simulink model "ex_kloss_startup"  (R2026b)
settings: Solver=ode23t  StopTime=2  MaxStep=1e-4  RelTol=1e-5
libraries: asm_blocks_lib x11, nesl_utility x1
settings Model: Creator=fsbb  LastModifiedBy=fsbb
settings SimscapeCC: SimscapeLogType=all  SimscapeNominalValues="[{\"value\":\"1\",\"unit\":\"A\"},{\"value\":\"1\",\"unit\":\"bar\"},{\"value\":\"1\",\"unit\":\"cm^2\"},{\"value\":\"1\",\"unit\":\"cm^3/s\"},{\"value\":\"1\",\"unit\":\"kJ/kg\"},{\"value\":\"1\",\"unit\":\"kW\"},{\"value\":\"1\",\"unit\":\"l\"},{\"value\":\"1\",\"unit\":\"N\"},{\"value\":\"1\",\"unit\":\"N*m\"},{\"value\":\"1\",\"unit\":\"V\"},{\"value\":\"0.001\",\"unit\":\"Wb\"}]"  SimscapeUseEnergyAccounting=off

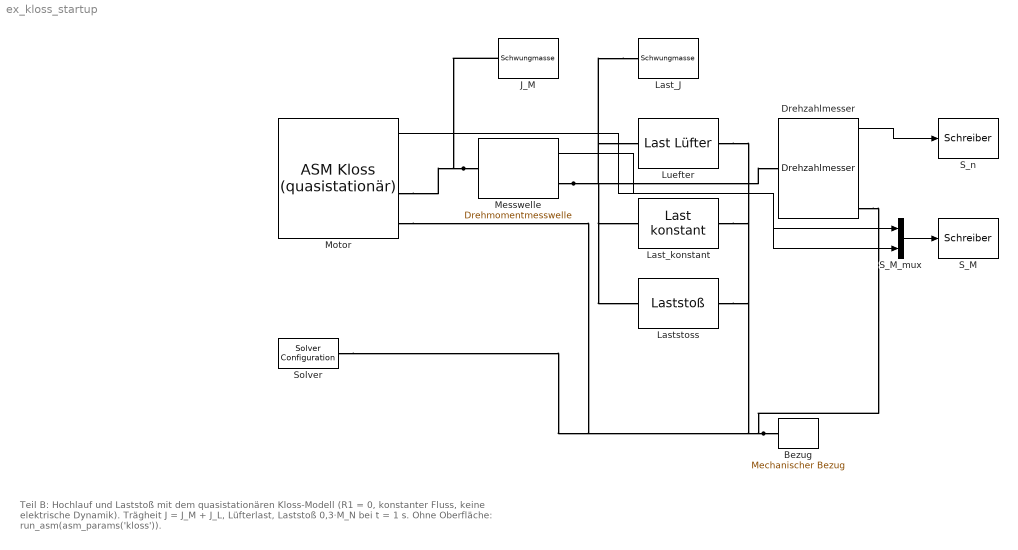
== system ex_kloss_startup ==
  note: Teil B: Hochlauf und Laststoß mit dem quasistationären Kloss-Modell (R1 = 0, konstanter Fluss, keine elektrische Dynamik). Trägheit J = J_M + J_L, Lüfterlast, Laststoß 0,3·M_N bei t = 1 s. Ohne Oberfläche: run_asm(asm_params('kloss')).
  Bezug : asm_blocks_lib/Mechanik/Mechanischer Bezug  Tag=asmlib:mech_reference
  Drehzahlmesser : asm_blocks_lib/Messgeräte/Drehzahlmesser  Tag=asmlib:speed_sensor  ns=1500
  J_M : asm_blocks_lib/Mechanik/Schwungmasse  Tag=asmlib:inertia  J=0.012  n0=0
  Last_J : asm_blocks_lib/Mechanik/Schwungmasse  Tag=asmlib:inertia  J=0.01  n0=0
  Last_konstant : asm_blocks_lib/Mechanik/Last konstant  Tag=asmlib:load_constant  M_L0=0
  Laststoss : asm_blocks_lib/Mechanik/Laststoß  Tag=asmlib:load_step  t_step=1  dM_L=7.95
  Luefter : asm_blocks_lib/Mechanik/Last Lüfter  Tag=asmlib:load_fan  M_B=26.5  n_B=1440
  Messwelle : asm_blocks_lib/Messgeräte/Drehmomentmesswelle  Tag=asmlib:torque_sensor
  Motor : asm_blocks_lib/Referenz/ASM Kloss (quasistationär)  Tag=asmlib:asm_kloss  MK=71.55  sK=0.2  ns=1500
  S_M : asm_blocks_lib/Messgeräte/Schreiber  Tag=asmlib:recorder  title_text=Motormoment (Kloss) und Wellenmoment
  S_M_mux : Mux  Inputs=2
  S_n : asm_blocks_lib/Messgeräte/Schreiber  Tag=asmlib:recorder  title_text=Drehzahl
  Solver : nesl_utility/Solver Configuration  PhysicalDomain=network_engine_domain  SubClassName=solver  LeftPortType=input  RightPortType=generic  Tones=[]  Harmonics=[]  SimulateNoise=off  Profile=off  UseLocalSampling=off  EnableSwitchedLinearOptims=on  FrequencyDomain=off  UseCCode=off  RelTol=0.001  AbsTol=0.001  MinStep=1e-09  ToWorkspace=off  RevertToSquareIcSolve=off  NumHomotopyIterations=100  PhasorMode=off  PhasorModeNumHarmonics=1  ConsistencySolver=NEWTON_XTOL_AFTER_FTOL  CanonicalOrdering=CANONICAL  OptimizeIntermediates=OPTIMIZED  MulticoreSolverChoice=BACKWARD_EULER  IndexReductionMethod=DerivativeReplacement  DoDC=off  ResidualTolerance=1e-09  ConsistencyTolSource=GLOBAL  ConsistencyAbsTol=0.001  ConsistencyRelTol=0.001  ConsistencyTolFactor=0.001  UseLocalSolver=off  LocalSolverChoice=NE_BACKWARD_EULER_ADVANCER  ResolveIndetEquations=on  FunctionEvalNumThread=1  LocalSolverSampleTime=0.001  DoFixedCost=off  MaxNonlinIter=3  MaxModeIter=2  ComputeImpulses=off  ImpulseIterations=2  LinearAlgebra=auto  LinearAlgebraNumThread=0  EquationFormulation=NE_TIME_EF  DelaysMemoryBudget=1024  AutomaticFiltering=on  FilteringTimeConstant=0.001  PartitionStorageMethod=AS_NEEDED  PartitionMemoryBudget=1024  PartitionMethod=BALANCED  MultibodyUseLocalSolver=off  MultibodyLocalSolverChoice=ODE1  MultibodyLocalSolverSampleTime=0.001
  wires:
  Drehzahlmesser/1 -> S_n/1
  Motor/1 -> S_M_mux/1
  Messwelle/1 -> S_M_mux/2
  S_M_mux/1 -> S_M/1
  connections:
  Messwelle/LConn1 -- Motor/RConn1 -- J_M/LConn1
  Motor/RConn2 -- Solver/RConn1 -- Luefter/RConn1 -- Last_konstant/RConn1 -- Laststoss/RConn1 -- Bezug/LConn1 -- Drehzahlmesser/RConn1
  Last_J/LConn1 -- Messwelle/RConn1 -- Luefter/LConn1 -- Last_konstant/LConn1 -- Laststoss/LConn1 -- Drehzahlmesser/LConn1
